simulink model "mars_rover_test_harness_chassis"  (R2025a)
settings: Solver=ode23t  StartTime=0.0  StopTime=30  FixedStep=1e-10  MaxStep=1e-1  RelTol=1e-3  AbsTol=1e-3  EnableMultiTasking=on
undefined symbols (not defined in the file): arm_q0, Control, L1, L2, L3, LS1, LS3, R1, R2, R3, Rover, RS1, RS3, X, Y, Z
libraries: sm_lib x119, nesl_utility x99, fl_lib x85, sdl_lib x20, ee_lib x10, mars_rover_lib x8, simulink x5, slpidlib x3, batteryecm_lib x2
(part 8 of 8)

== system mars_rover_test_harness_chassis/Rover/Chassis/Powertrain/Electrical/Steer/Sense tL3 ==
  Ideal Torque Sensor : fl_lib/Mechanical/Mechanical Sensors/Ideal Torque Sensor
  PS-Simulink Converter6 : nesl_utility/PS-Simulink Converter  PhysicalDomain=network_engine_domain  SubClassName=ps_output  LeftPortType=input  RightPortType=output  PseudoPeriodic=off  Frequencies=[]  VectorFormat=1-D array  Unit=inherit  AffineConversion=off
  C : PMIOPort  Side=Right
  R : PMIOPort  Port=2  Side=Left
  T : Outport
  wires:
  PS-Simulink Converter6/1 -> T/1
  connections:
  Ideal Torque Sensor/LConn1 -- R/RConn1
  Ideal Torque Sensor/RConn2 -- PS-Simulink Converter6/LConn1
  Ideal Torque Sensor/RConn1 -- C/RConn1

== system mars_rover_test_harness_chassis/Rover/Chassis/Powertrain/Electrical/Steer/Sense tR1 ==
  Ideal Torque Sensor : fl_lib/Mechanical/Mechanical Sensors/Ideal Torque Sensor
  PS-Simulink Converter6 : nesl_utility/PS-Simulink Converter  PhysicalDomain=network_engine_domain  SubClassName=ps_output  LeftPortType=input  RightPortType=output  PseudoPeriodic=off  Frequencies=[]  VectorFormat=1-D array  Unit=inherit  AffineConversion=off
  C : PMIOPort  Side=Right
  R : PMIOPort  Port=2  Side=Left
  T : Outport
  wires:
  PS-Simulink Converter6/1 -> T/1
  connections:
  Ideal Torque Sensor/RConn1 -- C/RConn1
  Ideal Torque Sensor/RConn2 -- PS-Simulink Converter6/LConn1
  Ideal Torque Sensor/LConn1 -- R/RConn1

== system mars_rover_test_harness_chassis/Rover/Chassis/Powertrain/Electrical/Steer/Sense tR3 ==
  Ideal Torque Sensor : fl_lib/Mechanical/Mechanical Sensors/Ideal Torque Sensor
  PS-Simulink Converter6 : nesl_utility/PS-Simulink Converter  PhysicalDomain=network_engine_domain  SubClassName=ps_output  LeftPortType=input  RightPortType=output  PseudoPeriodic=off  Frequencies=[]  VectorFormat=1-D array  Unit=inherit  AffineConversion=off
  C : PMIOPort  Side=Right
  R : PMIOPort  Port=2  Side=Left
  T : Outport
  wires:
  PS-Simulink Converter6/1 -> T/1
  connections:
  Ideal Torque Sensor/RConn1 -- C/RConn1
  Ideal Torque Sensor/RConn2 -- PS-Simulink Converter6/LConn1
  Ideal Torque Sensor/LConn1 -- R/RConn1

== system mars_rover_test_harness_chassis/Rover/Chassis/Powertrain/Electrical/Steer/Sensor iL1 ==
  Current Sensor : fl_lib/Electrical/Electrical Sensors/Current Sensor
  PS-Simulink Converter3 : nesl_utility/PS-Simulink Converter  PhysicalDomain=network_engine_domain  SubClassName=ps_output  LeftPortType=input  RightPortType=output  PseudoPeriodic=off  Frequencies=[]  VectorFormat=1-D array  Unit=inherit  AffineConversion=off
  + : PMIOPort  Side=Left
  - : PMIOPort  Port=2  Side=Right
  i : Outport
  wires:
  PS-Simulink Converter3/1 -> i/1
  connections:
  PS-Simulink Converter3/LConn1 -- Current Sensor/RConn1
  Current Sensor/RConn2 -- -/RConn1
  +/RConn1 -- Current Sensor/LConn1

== system mars_rover_test_harness_chassis/Rover/Chassis/Powertrain/Electrical/Steer/Sensor iL3 ==
  Current Sensor : fl_lib/Electrical/Electrical Sensors/Current Sensor
  PS-Simulink Converter3 : nesl_utility/PS-Simulink Converter  PhysicalDomain=network_engine_domain  SubClassName=ps_output  LeftPortType=input  RightPortType=output  PseudoPeriodic=off  Frequencies=[]  VectorFormat=1-D array  Unit=inherit  AffineConversion=off
  + : PMIOPort  Side=Left
  - : PMIOPort  Port=2  Side=Right
  i : Outport
  wires:
  PS-Simulink Converter3/1 -> i/1
  connections:
  +/RConn1 -- Current Sensor/LConn1
  Current Sensor/RConn2 -- -/RConn1
  PS-Simulink Converter3/LConn1 -- Current Sensor/RConn1

== system mars_rover_test_harness_chassis/Rover/Chassis/Powertrain/Electrical/Steer/Sensor iR1 ==
  Current Sensor : fl_lib/Electrical/Electrical Sensors/Current Sensor
  PS-Simulink Converter3 : nesl_utility/PS-Simulink Converter  PhysicalDomain=network_engine_domain  SubClassName=ps_output  LeftPortType=input  RightPortType=output  PseudoPeriodic=off  Frequencies=[]  VectorFormat=1-D array  Unit=inherit  AffineConversion=off
  + : PMIOPort  Side=Left
  - : PMIOPort  Port=2  Side=Right
  i : Outport
  wires:
  PS-Simulink Converter3/1 -> i/1
  connections:
  +/RConn1 -- Current Sensor/LConn1
  Current Sensor/RConn2 -- -/RConn1
  PS-Simulink Converter3/LConn1 -- Current Sensor/RConn1

== system mars_rover_test_harness_chassis/Rover/Chassis/Powertrain/Electrical/Steer/Sensor iR3 ==
  Current Sensor : fl_lib/Electrical/Electrical Sensors/Current Sensor
  PS-Simulink Converter3 : nesl_utility/PS-Simulink Converter  PhysicalDomain=network_engine_domain  SubClassName=ps_output  LeftPortType=input  RightPortType=output  PseudoPeriodic=off  Frequencies=[]  VectorFormat=1-D array  Unit=inherit  AffineConversion=off
  + : PMIOPort  Side=Left
  - : PMIOPort  Port=2  Side=Right
  i : Outport
  wires:
  PS-Simulink Converter3/1 -> i/1
  connections:
  PS-Simulink Converter3/LConn1 -- Current Sensor/RConn1
  Current Sensor/RConn2 -- -/RConn1
  +/RConn1 -- Current Sensor/LConn1

== system mars_rover_test_harness_chassis/Rover/Chassis/Powertrain/Ideal/Drive/Sense wL1 ==
  Ideal Rotational Motion Sensor : fl_lib/Mechanical/Mechanical Sensors/Ideal Rotational Motion Sensor  reference=foundation.enum.MeasurementReference.difference  acceleration_port=false  velocity_port=true  position_port=true  wrap_angle=simscape.enum.onoff.off  offset=0 rad
  PS Terminator : fl_lib/Physical Signals/Sinks/PS Terminator
  PS-Simulink Converter : nesl_utility/PS-Simulink Converter  PhysicalDomain=network_engine_domain  SubClassName=ps_output  LeftPortType=input  RightPortType=output  PseudoPeriodic=off  Frequencies=[]  VectorFormat=1-D array  Unit=inherit  AffineConversion=off
  R : PMIOPort  Side=Right
  C : PMIOPort  Port=2  Side=Left
  w : Outport
  wires:
  PS-Simulink Converter/1 -> w/1
  connections:
  Ideal Rotational Motion Sensor/RConn2 -- PS-Simulink Converter/LConn1
  Ideal Rotational Motion Sensor/LConn1 -- R/RConn1
  Ideal Rotational Motion Sensor/RConn1 -- C/RConn1
  Ideal Rotational Motion Sensor/RConn3 -- PS Terminator/LConn1

== system mars_rover_test_harness_chassis/Rover/Chassis/Powertrain/Ideal/Drive/Sense wL2 ==
  Ideal Rotational Motion Sensor : fl_lib/Mechanical/Mechanical Sensors/Ideal Rotational Motion Sensor  reference=foundation.enum.MeasurementReference.difference  acceleration_port=false  velocity_port=true  position_port=true  wrap_angle=simscape.enum.onoff.off  offset=0 rad
  PS Terminator : fl_lib/Physical Signals/Sinks/PS Terminator
  PS-Simulink Converter : nesl_utility/PS-Simulink Converter  PhysicalDomain=network_engine_domain  SubClassName=ps_output  LeftPortType=input  RightPortType=output  PseudoPeriodic=off  Frequencies=[]  VectorFormat=1-D array  Unit=inherit  AffineConversion=off
  R : PMIOPort  Side=Right
  C : PMIOPort  Port=2  Side=Left
  w : Outport
  wires:
  PS-Simulink Converter/1 -> w/1
  connections:
  Ideal Rotational Motion Sensor/RConn3 -- PS Terminator/LConn1
  Ideal Rotational Motion Sensor/RConn1 -- C/RConn1
  Ideal Rotational Motion Sensor/LConn1 -- R/RConn1
  Ideal Rotational Motion Sensor/RConn2 -- PS-Simulink Converter/LConn1

== system mars_rover_test_harness_chassis/Rover/Chassis/Powertrain/Ideal/Drive/Sense wL3 ==
  Ideal Rotational Motion Sensor : fl_lib/Mechanical/Mechanical Sensors/Ideal Rotational Motion Sensor  reference=foundation.enum.MeasurementReference.difference  acceleration_port=false  velocity_port=true  position_port=true  wrap_angle=simscape.enum.onoff.off  offset=0 rad
  PS Terminator : fl_lib/Physical Signals/Sinks/PS Terminator
  PS-Simulink Converter : nesl_utility/PS-Simulink Converter  PhysicalDomain=network_engine_domain  SubClassName=ps_output  LeftPortType=input  RightPortType=output  PseudoPeriodic=off  Frequencies=[]  VectorFormat=1-D array  Unit=inherit  AffineConversion=off
  R : PMIOPort  Side=Right
  C : PMIOPort  Port=2  Side=Left
  w : Outport
  wires:
  PS-Simulink Converter/1 -> w/1
  connections:
  Ideal Rotational Motion Sensor/RConn2 -- PS-Simulink Converter/LConn1
  Ideal Rotational Motion Sensor/LConn1 -- R/RConn1
  Ideal Rotational Motion Sensor/RConn1 -- C/RConn1
  Ideal Rotational Motion Sensor/RConn3 -- PS Terminator/LConn1

== system mars_rover_test_harness_chassis/Rover/Chassis/Powertrain/Ideal/Drive/Sense wR1 ==
  Ideal Rotational Motion Sensor : fl_lib/Mechanical/Mechanical Sensors/Ideal Rotational Motion Sensor  reference=foundation.enum.MeasurementReference.difference  acceleration_port=false  velocity_port=true  position_port=true  wrap_angle=simscape.enum.onoff.off  offset=0 rad
  PS Terminator : fl_lib/Physical Signals/Sinks/PS Terminator
  PS-Simulink Converter : nesl_utility/PS-Simulink Converter  PhysicalDomain=network_engine_domain  SubClassName=ps_output  LeftPortType=input  RightPortType=output  PseudoPeriodic=off  Frequencies=[]  VectorFormat=1-D array  Unit=inherit  AffineConversion=off
  R : PMIOPort  Side=Right
  C : PMIOPort  Port=2  Side=Left
  w : Outport
  wires:
  PS-Simulink Converter/1 -> w/1
  connections:
  Ideal Rotational Motion Sensor/RConn2 -- PS-Simulink Converter/LConn1
  Ideal Rotational Motion Sensor/LConn1 -- R/RConn1
  Ideal Rotational Motion Sensor/RConn1 -- C/RConn1
  Ideal Rotational Motion Sensor/RConn3 -- PS Terminator/LConn1

== system mars_rover_test_harness_chassis/Rover/Chassis/Powertrain/Ideal/Drive/Sense wR2 ==
  Ideal Rotational Motion Sensor : fl_lib/Mechanical/Mechanical Sensors/Ideal Rotational Motion Sensor  reference=foundation.enum.MeasurementReference.difference  acceleration_port=false  velocity_port=true  position_port=true  wrap_angle=simscape.enum.onoff.off  offset=0 rad
  PS Terminator : fl_lib/Physical Signals/Sinks/PS Terminator
  PS-Simulink Converter : nesl_utility/PS-Simulink Converter  PhysicalDomain=network_engine_domain  SubClassName=ps_output  LeftPortType=input  RightPortType=output  PseudoPeriodic=off  Frequencies=[]  VectorFormat=1-D array  Unit=inherit  AffineConversion=off
  R : PMIOPort  Side=Right
  C : PMIOPort  Port=2  Side=Left
  w : Outport
  wires:
  PS-Simulink Converter/1 -> w/1
  connections:
  Ideal Rotational Motion Sensor/RConn3 -- PS Terminator/LConn1
  Ideal Rotational Motion Sensor/RConn1 -- C/RConn1
  Ideal Rotational Motion Sensor/LConn1 -- R/RConn1
  Ideal Rotational Motion Sensor/RConn2 -- PS-Simulink Converter/LConn1

== system mars_rover_test_harness_chassis/Rover/Chassis/Powertrain/Ideal/Drive/Sense wR3 ==
  Ideal Rotational Motion Sensor : fl_lib/Mechanical/Mechanical Sensors/Ideal Rotational Motion Sensor  reference=foundation.enum.MeasurementReference.difference  acceleration_port=false  velocity_port=true  position_port=true  wrap_angle=simscape.enum.onoff.off  offset=0 rad
  PS Terminator : fl_lib/Physical Signals/Sinks/PS Terminator
  PS-Simulink Converter : nesl_utility/PS-Simulink Converter  PhysicalDomain=network_engine_domain  SubClassName=ps_output  LeftPortType=input  RightPortType=output  PseudoPeriodic=off  Frequencies=[]  VectorFormat=1-D array  Unit=inherit  AffineConversion=off
  R : PMIOPort  Side=Right
  C : PMIOPort  Port=2  Side=Left
  w : Outport
  wires:
  PS-Simulink Converter/1 -> w/1
  connections:
  Ideal Rotational Motion Sensor/RConn2 -- PS-Simulink Converter/LConn1
  Ideal Rotational Motion Sensor/LConn1 -- R/RConn1
  Ideal Rotational Motion Sensor/RConn1 -- C/RConn1
  Ideal Rotational Motion Sensor/RConn3 -- PS Terminator/LConn1

== system mars_rover_test_harness_chassis/Rover/Chassis/Powertrain/Ideal/Power/Sensing Temperature ==
  PS-Simulink Converter : nesl_utility/PS-Simulink Converter  PhysicalDomain=network_engine_domain  SubClassName=ps_output  LeftPortType=input  RightPortType=output  PseudoPeriodic=off  Frequencies=[]  VectorFormat=1-D array  Unit=inherit  AffineConversion=off
  Temperature Sensor : fl_lib/Thermal/Thermal Sensors/Temperature Sensor  temperature_measure=foundation.enum.MeasurementReference.difference
  Thermal Reference : fl_lib/Thermal/Thermal Elements/Thermal Reference
  A : PMIOPort  Side=Left
  T : Outport
  wires:
  PS-Simulink Converter/1 -> T/1
  connections:
  Thermal Reference/LConn1 -- Temperature Sensor/RConn1
  Temperature Sensor/RConn2 -- PS-Simulink Converter/LConn1
  A/RConn1 -- Temperature Sensor/LConn1

== system mars_rover_test_harness_chassis/Rover/Chassis/Powertrain/Ideal/Steer/Sense wL1 ==
  Ideal Rotational Motion Sensor : fl_lib/Mechanical/Mechanical Sensors/Ideal Rotational Motion Sensor  reference=foundation.enum.MeasurementReference.difference  acceleration_port=false  velocity_port=true  position_port=true  wrap_angle=simscape.enum.onoff.off  offset=0 rad
  PS Terminator : fl_lib/Physical Signals/Sinks/PS Terminator
  PS-Simulink Converter : nesl_utility/PS-Simulink Converter  PhysicalDomain=network_engine_domain  SubClassName=ps_output  LeftPortType=input  RightPortType=output  PseudoPeriodic=off  Frequencies=[]  VectorFormat=1-D array  Unit=inherit  AffineConversion=off
  R : PMIOPort  Side=Right
  C : PMIOPort  Port=2  Side=Left
  w : Outport
  wires:
  PS-Simulink Converter/1 -> w/1
  connections:
  Ideal Rotational Motion Sensor/RConn2 -- PS-Simulink Converter/LConn1
  Ideal Rotational Motion Sensor/LConn1 -- R/RConn1
  Ideal Rotational Motion Sensor/RConn1 -- C/RConn1
  Ideal Rotational Motion Sensor/RConn3 -- PS Terminator/LConn1

== system mars_rover_test_harness_chassis/Rover/Chassis/Powertrain/Ideal/Steer/Sense wL3 ==
  Ideal Rotational Motion Sensor : fl_lib/Mechanical/Mechanical Sensors/Ideal Rotational Motion Sensor  reference=foundation.enum.MeasurementReference.difference  acceleration_port=false  velocity_port=true  position_port=true  wrap_angle=simscape.enum.onoff.off  offset=0 rad
  PS Terminator : fl_lib/Physical Signals/Sinks/PS Terminator
  PS-Simulink Converter : nesl_utility/PS-Simulink Converter  PhysicalDomain=network_engine_domain  SubClassName=ps_output  LeftPortType=input  RightPortType=output  PseudoPeriodic=off  Frequencies=[]  VectorFormat=1-D array  Unit=inherit  AffineConversion=off
  R : PMIOPort  Side=Right
  C : PMIOPort  Port=2  Side=Left
  w : Outport
  wires:
  PS-Simulink Converter/1 -> w/1
  connections:
  Ideal Rotational Motion Sensor/RConn2 -- PS-Simulink Converter/LConn1
  Ideal Rotational Motion Sensor/LConn1 -- R/RConn1
  Ideal Rotational Motion Sensor/RConn1 -- C/RConn1
  Ideal Rotational Motion Sensor/RConn3 -- PS Terminator/LConn1

== system mars_rover_test_harness_chassis/Rover/Chassis/Powertrain/Ideal/Steer/Sense wR1 ==
  Ideal Rotational Motion Sensor : fl_lib/Mechanical/Mechanical Sensors/Ideal Rotational Motion Sensor  reference=foundation.enum.MeasurementReference.difference  acceleration_port=false  velocity_port=true  position_port=true  wrap_angle=simscape.enum.onoff.off  offset=0 rad
  PS Terminator : fl_lib/Physical Signals/Sinks/PS Terminator
  PS-Simulink Converter : nesl_utility/PS-Simulink Converter  PhysicalDomain=network_engine_domain  SubClassName=ps_output  LeftPortType=input  RightPortType=output  PseudoPeriodic=off  Frequencies=[]  VectorFormat=1-D array  Unit=inherit  AffineConversion=off
  R : PMIOPort  Side=Right
  C : PMIOPort  Port=2  Side=Left
  w : Outport
  wires:
  PS-Simulink Converter/1 -> w/1
  connections:
  Ideal Rotational Motion Sensor/RConn2 -- PS-Simulink Converter/LConn1
  Ideal Rotational Motion Sensor/LConn1 -- R/RConn1
  Ideal Rotational Motion Sensor/RConn1 -- C/RConn1
  Ideal Rotational Motion Sensor/RConn3 -- PS Terminator/LConn1

== system mars_rover_test_harness_chassis/Rover/Chassis/Powertrain/Ideal/Steer/Sense wR3 ==
  Ideal Rotational Motion Sensor : fl_lib/Mechanical/Mechanical Sensors/Ideal Rotational Motion Sensor  reference=foundation.enum.MeasurementReference.difference  acceleration_port=false  velocity_port=true  position_port=true  wrap_angle=simscape.enum.onoff.off  offset=0 rad
  PS Terminator : fl_lib/Physical Signals/Sinks/PS Terminator
  PS-Simulink Converter : nesl_utility/PS-Simulink Converter  PhysicalDomain=network_engine_domain  SubClassName=ps_output  LeftPortType=input  RightPortType=output  PseudoPeriodic=off  Frequencies=[]  VectorFormat=1-D array  Unit=inherit  AffineConversion=off
  R : PMIOPort  Side=Right
  C : PMIOPort  Port=2  Side=Left
  w : Outport
  wires:
  PS-Simulink Converter/1 -> w/1
  connections:
  Ideal Rotational Motion Sensor/RConn2 -- PS-Simulink Converter/LConn1
  Ideal Rotational Motion Sensor/LConn1 -- R/RConn1
  Ideal Rotational Motion Sensor/RConn1 -- C/RConn1
  Ideal Rotational Motion Sensor/RConn3 -- PS Terminator/LConn1

== matlab function mars_rover_test_harness_chassis/Control/Chassis Control/Ackerman Steer Angle/Ackerman Steering Angle Formulation ==
  data: delta input; qSteerL3 output; L input; qSteerR3 output; d input; R output; L_R output; R_R output
function [qSteerL3,qSteerR3,R,L_R,R_R] = fcn(delta,L,d)
% Function to compute ackerman steering angles 
% from a bicycle steer angle.

R = L/tand(abs(delta));

if delta < 0
    qSteerL3 = atan2d(L,(R+d/2));
    qSteerR3 = atan2d(L,(R-d/2));
    L_R = (R+d/2);
    R_R = (R-d/2);
else
    qSteerL3 = -atan2d(L,(R-d/2));
    qSteerR3 = -atan2d(L,(R+d/2));
    L_R = (R-d/2);
    R_R = (R+d/2);
end

end

== matlab function mars_rover_test_harness_chassis/Control/Chassis Control/Chassis Velocity To Wheel Speed ==
  data: vTarget input; steer_ang input; A3_ROC input; L3_ROC input; R3_ROC input; wL1 output; wheel_r input; wL2 output; wL3 output; L input; wR1 output; wR2 output; wR3 output
function [wL1,wL2,wL3, wR1,wR2,wR3] = ...
    fcn(vTarget,steer_ang,A3_ROC,L3_ROC,R3_ROC,wheel_r,L)
% Function to compute wheel speed from a desired linear velocity and
% desired path.

if any(abs(steer_ang) > 0)

    wL1 = (vTarget/wheel_r)*sqrt(L3_ROC^2 + L^2)/A3_ROC;
    wL2 = vTarget * L3_ROC/(A3_ROC*wheel_r);
    wL3 = (vTarget/wheel_r)*sqrt(L3_ROC^2 + L^2)/A3_ROC;
    wR1 = (vTarget/wheel_r)*sqrt(R3_ROC^2 + L^2)/A3_ROC;
    wR2 = vTarget * R3_ROC/(A3_ROC*wheel_r);
    wR3 = (vTarget/wheel_r)*sqrt(R3_ROC^2 + L^2)/A3_ROC;

else
    wL1 = vTarget / wheel_r;
    wL2 = vTarget / wheel_r;
    wL3 = vTarget / wheel_r;
    wR1 = vTarget / wheel_r;
    wR2 = vTarget / wheel_r;
    wR3 = vTarget / wheel_r;
end

end
